simulink model "test_on_proxy"  (R2025b)
settings: Solver=FixedStepAuto  StartTime=0.0  StopTime=91  FixedStep=0.001  RelTol=1e-3
undefined symbols (not defined in the file): DiscIntNeverNeededParam, Ts, x0_eq
libraries: eeGeneralControl x1
(part 2 of 2)

== matlab function test_on_proxy/mpc_core_codegen2 ==
  data: theta_meas input; omega_meas input; eps_center_total_meas input; eps_center_dyn_meas input; theta_ref input; x_prev input; Jrig input; Brig input; max_angle input; Qth input; QtipVel input; Qbend input; Qq_base input; Qv_base input; umax input; du_rate_max input; Sdu input; Ru input; m_payload input; m_payload_step input; gravity_sign input; gravity_correction input; use_gravity_compensation input; zeta input; tol input; S_theta_base input; S_theta_high input; terminal_cost_gain_base input; terminal_law_gain_base input; term_gain_min input; term_gain_max input; S_term_box input; uNm output; u_mpc output; x_next output; y_geom output; y_rate output; EPS_my output; y_rate_mpc output; m_proj_base output; tau_g_ff output; offset_based_geom_angle output; terminal_cost_value output; terminal_error_norm output; terminal_u_lqr output; terminal_u_last output; terminal_u_match_error output; terminal_inside_flag output; terminal_lyap_delta output; terminal_cost_ratio output; alpha_term_vis output; terminal_cost_normalized output; terminal_inside_flag_strict output; terminal_inside_flag_soft output; terminal_set_slack output; terminal_set_box_violation output; z_out output; g_dyn output; x_hat output
function [uNm,u_mpc, x_next, y_geom, y_rate, EPS_my, y_rate_mpc, ...
          m_proj_base,tau_g_ff,offset_based_geom_angle, ...
          terminal_cost_value, terminal_error_norm, ...
          terminal_u_lqr, terminal_u_last, terminal_u_match_error, ...
          terminal_inside_flag, terminal_lyap_delta, ...
          terminal_cost_ratio, alpha_term_vis, ...
          terminal_cost_normalized, terminal_inside_flag_strict, terminal_inside_flag_soft, ...
          terminal_set_slack, terminal_set_box_violation,z_out,g_dyn,x_hat]  = mpc_core_codegen( ...
    theta_meas, omega_meas, ...
    eps_center_total_meas, ...
    eps_center_dyn_meas, ...
    theta_ref, x_prev,Jrig,Brig, ...
    max_angle,Qth,QtipVel,Qbend,Qq_base,Qv_base,umax,du_rate_max,Sdu,Ru,...
    m_payload,m_payload_step,gravity_sign,gravity_correction,use_gravity_compensation,...
    zeta,tol,S_theta_base,S_theta_high,...
    terminal_cost_gain_base,terminal_law_gain_base,term_gain_min,term_gain_max,S_term_box) %#codegen

NM = coder.const(1);                      % only 1 flex mode used
NX = coder.const(2 + 2*NM);              % x = [theta omega q v]
NY = coder.const(3 + 2*NM);              % y = [geom bend tiprate q v]
NP = coder.const(65);                    % prediction horizon
NC = coder.const(13);                    % control horizon
NS = coder.const(min(100, 60*NM));       % spatial integration points

Nm = NM; nx = NX; ny = NY; Np = NP; Nc = NC; Ns = NS;

persistent zeta_ref omega_ref init_zeta_ref
persistent last_m_payload_model

persistent L b  h E rho Izz EI Acs yb

persistent init_done
persistent Ts iy_geom iy_tipdot iy_bend
persistent m_beam
persistent g

persistent Ad Bd Taff Cd_static
persistent s Alpha aL dphiL Phi_hat rhoA Minv Minv_c
persistent Sx Su_base Su Qz w_trap

persistent u_prev dU_prev
persistent k_strain
persistent phi_tip_hat
persistent J_tip_eff

persistent buf_xa buf_yoff buf_Crow buf_q
persistent idx_qi idx_vi
persistent umax_stack dumax_vec

persistent pw_vec_ext
persistent max_iter

persistent theta_max
persistent M_con

persistent xnom_all Crow_all yoff_nom_all
persistent Fi_all Gi_all
persistent Gabs Ginc QGinc
persistent onesNc

persistent Pterm Kterm Cd_term0 Crow_term0
persistent alpha_term
persistent alpha_vis_scale
persistent theta_ref_clip_margin

persistent term_box

% --- persistents for total/dynamic epsilon handling ---
persistent q_total_filt_prev
persistent q_dyn_prev
persistent alpha_q_total
payload_step_eff = max(abs(m_payload_step), 1e-9);
if m_payload >= 0.1
   m_payload = 0; 
    
end
m_payload_model  = payload_step_eff * round(m_payload / payload_step_eff);

% ============================================================
% First-time fixed initialization
% ============================================================
if isempty(init_done)

  
    L   = 0.5;                            % beam length
    b   = 0.02;                           % beam width
    h   = 0.002;                          % beam thickness
    E   = 70e9;
    rho = 2755;
    Acs = b*h;
    Izz = b*h^3/12;
    EI  = E*Izz;
    rhoA = rho*Acs;                       % mass per length
    yb  = 0.5*h;                          % outer fiber distance for strain relation

    fs = 1000;
    Ts = 1/fs;

    g = 9.81;

     theta_max = max_angle * pi/180;
    M_con     = min(Np,15);
    max_iter  = 60;

    m_beam = rhoA * L;

    s = linspace(0,L,Ns).';

    w_trap = zeros(Ns,1);
    for i = 2:Ns
        hseg = s(i) - s(i-1);
        w_trap(i-1) = w_trap(i-1) + 0.5*hseg;
        w_trap(i)   = w_trap(i)   + 0.5*hseg;
    end

    iy_geom   = 1;
    iy_bend   = 2;
    iy_tipdot = 3;

    Qdiag = zeros(ny,1);
    Qdiag(iy_geom)   = Qth;
    Qdiag(iy_bend)   = Qbend;
    Qdiag(iy_tipdot) = QtipVel;

    rowQ = 3;
    for i = 1:Nm
        Qdiag(rowQ+i) = Qq_base;
    end

    rowV = 3 + Nm;
    for i = 1:Nm
        Qdiag(rowV+i) = Qv_base;
    end

    Qz = diag(Qdiag);

    u_prev  = 0;
    dU_prev = zeros(Nc,1);

    buf_xa   = zeros(nx,1);
    buf_yoff = zeros(ny,1);
    buf_Crow = zeros(1,nx);
    buf_q    = zeros(Nm,1);

    idx_qi = zeros(Nm,1);
    idx_vi = zeros(Nm,1);
    for i = 1:Nm
        idx_qi(i) = 2 + 2*(i-1) + 1;
        idx_vi(i) = idx_qi(i) + 1;
    end

    umax_stack = umax*ones(Nc,1);
    dumax_vec  = du_rate_max*ones(Nc,1);

    pw_vec_ext = ones(Nc+2,1) / sqrt(Nc+2);

    xnom_all      = zeros(nx,Np);
    Crow_all      = zeros(Np,nx);
    yoff_nom_all  = zeros(Np,1);
    Fi_all        = zeros(ny,Np);
    Gi_all        = zeros(ny,Nc,Np);

    Gabs  = zeros(ny,Nc);
    Ginc  = zeros(ny,Nc);
    QGinc = zeros(ny,Nc);

    onesNc = ones(Nc,1);

    alpha_vis_scale = 1.0;
    theta_ref_clip_margin = 0.5*pi/180.0;

    term_box = zeros(nx,1);
    term_box(1) = 40*pi/180.0;
    term_box(2) = 80*pi/180.0;
    term_box(3) = 1;
    term_box(4) = 1.0;

    q_dyn_prev         = 0.0;
    q_total_filt_prev  = 0.0;
    alpha_q_total      = 0.10;

    last_m_payload_model = -1e99;

    % =========================
    % NEW: initialize zeta reference
    % =========================
    init_zeta_ref = false;
    omega_ref = zeros(Nm,1);
    zeta_ref  = zeta;
end

% ============================================================
% Payload-dependent model rebuild
% ============================================================
if abs(m_payload_model - last_m_payload_model) > 1e-12 || isempty(init_done)

    M_phi   = m_payload_model;
    M_mass  = m_payload_model;
    M_betaL = m_payload_model;
    J_tip_eff = 0.0;

    betaL = compute_payload_roots(Nm, rhoA, EI, L, M_betaL, J_tip_eff);

    omega_n = zeros(Nm,1);
    scale_omega = sqrt(EI / rhoA) / (L^2);
    for i = 1:Nm
        omega_n(i) = (betaL(i)^2) * scale_omega;
    end

    z = zeros(Nm,1);

    Phi      = zeros(Ns,Nm);
    Alpha    = zeros(Ns,Nm);
    dphiL    = zeros(Nm,1);
    phi_tip_hat = zeros(Nm,1);

    for i = 1:Nm

        phi_raw  = payload_shape(betaL(i), L, s, rhoA, M_phi);
        dphi_raw = payload_shape_d(betaL(i), L, s, rhoA, M_phi);

        phi_tip = payload_shape(betaL(i), L, L, rhoA, M_phi);
        sc = 1 / max(abs(phi_tip), 1e-12);

        phi_raw  = phi_raw  * sc;
        dphi_raw = dphi_raw * sc;

        % =========================
        % Modal mass FULL
        % =========================
        m_eff_beam = dot(w_trap, rhoA*(phi_raw.^2));

        m_eff_payload = M_mass*(phi_raw(end)^2) ...
                      + J_tip_eff*(dphi_raw(end)^2);

        m_eff_total = m_eff_beam + m_eff_payload;

        % normalization
        cn = 1 / sqrt(max(m_eff_total,1e-12));

        % =========================
        % NEW: ZETA UPDATE WITH PAYLOAD
        % =========================
        % First model rebuild stores reference omega and zeta.
        % Later, when payload changes omega_n, zeta is updated so that:
        %
        %   2*zeta_new*omega_new = 2*zeta_ref*omega_ref
        %
        % This keeps the modal damping coefficient approximately constant.

        if ~init_zeta_ref
            zeta_ref  = zeta;
            omega_ref = omega_n;
            init_zeta_ref = true;
        end

        zeta_eff_i = zeta_ref * omega_ref(i) / max(omega_n(i),1e-12);

        % safety clamp
        zeta_eff_i = clamp_scalar(zeta_eff_i, 1e-5, 0.5);

        z(i) = zeta_eff_i;

        % =========================
        % STORE MODES
        % =========================
        Phi(:,i)       = phi_raw;
        Alpha(:,i)     = cn * dphi_raw;
        dphiL(i)       = cn * dphi_raw(end);
        phi_tip_hat(i) = cn * phi_raw(end);
    end

    Phi_hat = zeros(Ns,Nm);
    for i = 1:Nm
        phi_raw  = payload_shape(betaL(i), L, s, rhoA, M_phi);
        dphi_raw = payload_shape_d(betaL(i), L, s, rhoA, M_phi);
        phi_tip  = payload_shape(betaL(i), L, L, rhoA, M_phi);

        sc = 1 / max(abs(phi_tip), 1e-12);

        phi_raw  = phi_raw  * sc;
        dphi_raw = dphi_raw * sc;

        mi_loc = dot(w_trap, rhoA*(phi_raw.^2)) ...
               + M_mass*(phi_raw(end)^2) ...
               + J_tip_eff*(dphi_raw(end)^2);

        cn = 1 / sqrt(max(mi_loc,1e-12));

        Phi_hat(:,i)    = cn * phi_raw;
        Alpha(:,i)      = cn * dphi_raw;
        dphiL(i)        = cn * dphi_raw(end);
        phi_tip_hat(i)  = cn * phi_raw(end);
    end

    c_base = zeros(Nm,1);
    for i = 1:Nm
        c_base(i) = dot(w_trap, rhoA*(s .* Phi_hat(:,i))) ...
                  + M_mass * L * phi_tip_hat(i);
    end

    Mmod = eye(Nm);
    Kmod = diag(omega_n.^2);
    Dmod = diag(2*z(:).*omega_n(:));
    Minv = inv(Mmod);

    aL     = Alpha(end,:).';
    Minv_c = Minv * c_base;

    A = zeros(nx);
    B = zeros(nx,1);

    A(1,2) = 1;
    A(2,2) = -(Brig/Jrig);
    B(2,1) = 1/Jrig;

    Aqq = -Minv*Kmod;
    Avv = -Minv*Dmod;

    for i = 1:Nm
        qi = idx_qi(i);
        vi = idx_vi(i);

        A(qi,vi) = 1;

        for j = 1:Nm
            qj = idx_qi(j);
            vj = idx_vi(j);

            A(vi,qj) = A(vi,qj) + Aqq(i,j);
            A(vi,vj) = A(vi,vj) + Avv(i,j);
        end

        B(vi,1) = B(vi,1) - (1/Jrig)*Minv_c(i);
        A(vi,2) = A(vi,2) + (Brig/Jrig)*Minv_c(i);
    end

    [Ad,Bd,Taff] = c2d_expm_affine_vec(A,B,Ts);

    Cd_static = zeros(ny,nx);

    Cd_static(iy_tipdot,2) = 1;
    for i = 1:Nm
        vi = idx_vi(i);
        Cd_static(iy_tipdot,vi) = Cd_static(iy_tipdot,vi) + dphiL(i);
    end

    for i = 1:Nm
        qi = idx_qi(i);
        Cd_static(iy_bend,qi) = Cd_static(iy_bend,qi) + 1.0;
    end

    rowQ = 3;
    for i = 1:Nm
        Cd_static(rowQ+i, idx_qi(i)) = 1;
    end

    rowV = 3 + Nm;
    for i = 1:Nm
        Cd_static(rowV+i, idx_vi(i)) = 1;
    end

    [Sx,Su_base,Su] = precompute_prediction_scaffolds_fast(Ad,Bd,Np,Nc,nx);

    sensor_s = 0.05;
    k_strain = zeros(Nm,1);

    for i = 1:Nm
        phi_dd_i = payload_shape_dd(betaL(i), L, sensor_s, rhoA, M_phi);

        phi_tip  = payload_shape(betaL(i), L, L, rhoA, M_phi);
        sc       = 1 / max(abs(phi_tip), 1e-12);
        phi_dd_i = phi_dd_i * sc;

        dphi_raw = payload_shape_d(betaL(i), L, s, rhoA, M_phi) * sc;
        phi_raw  = payload_shape(betaL(i), L, s, rhoA, M_phi) * sc;

        mi_loc = dot(w_trap, rhoA*(phi_raw.^2)) ...
               + M_mass*(phi_raw(end)^2) ...
               + J_tip_eff*(dphi_raw(end)^2);

        cn = 1 / sqrt(max(mi_loc,1e-12));

        k_strain(i) = yb * cn * phi_dd_i;
    end

    xeq_term0 = zeros(nx,1);
    qtmp_term = zeros(Nm,1);
    Crow_tmp  = zeros(1,nx);

    [~, Crow_term0, ~] = chord_angle_and_jac_analytic( ...
        xeq_term0, Alpha, w_trap, Nm, qtmp_term, Crow_tmp);

    Cd_term0 = Cd_static;
    Cd_term0(iy_geom,:) = Crow_term0;

    Qx_term = zeros(nx,nx);
    Qx_term(1,1) = 1.0;
    Qx_term(2,2) = 0.5;
    Qx_term(3,3) = 0.2;
    Qx_term(4,4) = 0.1;

    [Pterm, Kterm] = dlqr_terminal_design_iter(Ad, Bd, Qx_term, max(Ru,1e-3));

    u_term_max     = umax;
    theta_term_max = theta_max;

    denom_u = Kterm * (Pterm \ Kterm.');
    if denom_u < 1e-12
        denom_u = 1e-12;
    end
    alpha_u = (u_term_max^2) / denom_u;

    hth = Crow_term0;
    denom_th = hth * (Pterm \ hth.');
    if denom_th < 1e-12
        denom_th = 1e-12;
    end
    alpha_th = (theta_term_max^2) / denom_th;

    alpha_term = min(alpha_u, alpha_th);
    init_done = true;
    last_m_payload_model = m_payload_model;
end

terminal_cost_value    = 0.0;
terminal_error_norm    = 0.0;
terminal_u_lqr         = 0.0;
terminal_u_last        = 0.0;
terminal_u_match_error = 0.0;
terminal_inside_flag   = 0.0;
terminal_lyap_delta    = 0.0;
terminal_cost_ratio    = 0.0;
alpha_term_vis         = alpha_vis_scale * alpha_term;
terminal_cost_normalized = 0.0;
terminal_inside_flag_strict = 0.0;
terminal_inside_flag_soft   = 0.0;
terminal_set_slack = 0.0;
terminal_set_box_violation = 0.0;

% -------------------------------------------------------------------------
% STATE RECONSTRUCTION
% -------------------------------------------------------------------------
x_hat = x_prev;
x_hat(1) = theta_meas;
x_hat(2) = omega_meas;

if isempty(q_dyn_prev)
   q_dyn_prev = x_hat(3);
end

% dynamic epsilon -> dynamic q/v used by controller
q_dyn_meas = eps_center_dyn_meas / k_strain(1);
v_dyn_raw  = (q_dyn_meas - q_dyn_prev) / Ts;
q_dyn_prev = q_dyn_meas;

% total epsilon -> full-bend monitor only
q_total_meas = eps_center_total_meas / k_strain(1);
q_total_now  = (1.0 - alpha_q_total)*q_total_filt_prev + alpha_q_total*q_total_meas;

% IMPORTANT:
% Controller state must use consistent q and v.
% Do not mix total q with dynamic v.
x_hat(3) = q_total_meas;
x_hat(4) = -v_dyn_raw;

q_total_filt_prev = q_total_now;

buf_xa(:) = x_hat;
xa = buf_xa;

% reconstructed total strain monitor
EPS_my = k_strain(1) * q_total_now;

% use total epsilon-based bend proxy only for offset-based monitor
offset_theoretical = -(0.5^3*EPS_my)/(3*(0.5-0.05)*0.5*0.002) ...
                   + (0.5405*0.5^2*cos(xa(1)))/(24*70e9*0.02*0.002^3/12)*(0.5-4*0.05);

x_Hafsa = cos(xa(1)) - offset_theoretical*sin(xa(1));
y_Hafsa = sin(xa(1)) - offset_theoretical*cos(xa(1));
offset_based_geom_angle = atan2(y_Hafsa,x_Hafsa);

[thg, Crow_now, y_off_now] = chord_angle_and_jac_analytic( ...
    xa, Alpha, w_trap, Nm, buf_q, buf_Crow);

Cd_now = Cd_static;
Cd_now(iy_geom,:) = Crow_now;

yoff_now = buf_yoff;
yoff_now(:) = 0;
yoff_now(iy_geom) = y_off_now;

y_now      = Cd_now*xa + yoff_now;
y_rate_mpc = y_now(iy_tipdot);

theta_ref_eff = clamp_scalar(theta_ref, -(theta_max - theta_ref_clip_margin), (theta_max - theta_ref_clip_margin));

dist_theta = theta_max - abs(thg);
if dist_theta < 10*pi/180
    S_theta = S_theta_high;
else
    S_theta = S_theta_base;
end

% -------------------------------------------------------------------------
% TERMINAL TARGET
% use pure zero-flex terminal target because dynamic epsilon is dynamic-only
% -------------------------------------------------------------------------
xeq_term = zeros(nx,1);
xeq_term(1) = theta_ref_eff;
xeq_term(2) = 0.0;
xeq_term(3) = 0.0;
xeq_term(4) = 0.0;

[tau_eq_ff, ~] = gravity_torque_ff_from_state( ...
    xeq_term, s, Alpha, gravity_sign, g, rhoA, m_payload, Nm, idx_qi);

u_eq_term = tau_eq_ff * use_gravity_compensation + gravity_correction;
u_eq_term = clamp_scalar(u_eq_term, -umax, umax);

x_nom = xa;
for i = 1:Np
    [g_dyn_nom, ~, ~] = gravity_vector_from_state( ...
        x_nom, Alpha, aL, w_trap, rhoA, Phi_hat, phi_tip_hat, Minv, ...
        gravity_sign, g, m_payload, Nm, nx, idx_qi, idx_vi);

    x_nom = Ad*x_nom + Bd*u_prev + Taff*g_dyn_nom;
    xnom_all(:,i) = x_nom;

    [~, Crow_i, yoff_i] = chord_angle_and_jac_analytic( ...
        x_nom, Alpha, w_trap, Nm, buf_q, buf_Crow);

    Crow_all(i,:)     = Crow_i;
    yoff_nom_all(i,1) = yoff_i;
end

rowsN = (Np-1)*nx + (1:nx);
GxN   = Su_base(rowsN,1:Nc) * Su;
xNnom = xnom_all(:,Np);
eNnom = xNnom - xeq_term;

term_metric_nom = eNnom.' * Pterm * eNnom;
term_ratio_nom  = term_metric_nom / max(alpha_term,1e-12);

term_sched = 1.0 / (1.0 + term_ratio_nom);
term_sched = clamp_scalar(term_sched, term_gain_min, term_gain_max);

terminal_cost_gain = terminal_cost_gain_base * term_sched;
terminal_law_gain  = terminal_law_gain_base  * term_sched;

H_base = zeros(Nc,Nc);
f_base = zeros(Nc,1);

for i = 1:Np
    rows_x = (i-1)*nx + (1:nx);
    mi_h = min(i, Nc);

    Cd_i = Cd_static;
    Cd_i(iy_geom,:) = Crow_all(i,:);

    Fi = Cd_i * xnom_all(:,i);

    Gabs(:,:) = Cd_i * Su_base(rows_x,1:Nc);
    Ginc(:,:) = Gabs * Su;

    for k = 1:Nc
        if k > mi_h
            for r = 1:ny
                Ginc(r,k) = 0;
            end
        end
    end

    QGinc(:,:) = Qz * Ginc;
    H_base = H_base + Ginc.' * QGinc;

    yi = Fi;
    yi(iy_geom) = yi(iy_geom) + yoff_nom_all(i) - theta_ref_eff;

    f_base = f_base + Ginc.' * (Qz * yi);

    Fi_all(:,i)   = Fi;
    Gi_all(:,:,i) = Ginc;
end

H_base = H_base + terminal_cost_gain * (GxN.' * Pterm * GxN);
f_base = f_base + terminal_cost_gain * (GxN.' * (Pterm * eNnom));

Su_last = zeros(1,Nc);
for k = 1:Nc
    Su_last(k) = 1.0;
end

a_term = Su_last - Kterm * GxN;
b_term = (Kterm * eNnom) + u_eq_term - u_prev;

H_base = H_base + terminal_law_gain * (a_term.' * a_term);
f_base = f_base - terminal_law_gain * (a_term.' * b_term);

H_base = H_base + (Ru * (Su.' * Su)) + Sdu*eye(Nc);
f_base = f_base + Ru * (Su.' * (u_prev * onesNc));

H_base = 0.5*(H_base + H_base.');

nU         = Nc;
nSlackAng  = 1;
nSlackTerm = 1;
nZ         = nU + nSlackAng + nSlackTerm;

idx_ang_slack  = nU + 1;
idx_term_slack = nU + 2;

H_ext = zeros(nZ,nZ);
H_ext(1:nU,1:nU) = H_base;
H_ext(idx_ang_slack,idx_ang_slack)  = 2*S_theta;
H_ext(idx_term_slack,idx_term_slack)= 2*S_term_box;

f_ext       = zeros(nZ,1);
f_ext(1:nU) = f_base;

Nlin   = 2*M_con + 1 + 2*nx + 1;
A_ineq = zeros(Nlin, nZ);
b_ineq = zeros(Nlin, 1);
row_idx = 0;

for i = 1:M_con
    Fi_i   = Fi_all(:,i);
    Gi_i   = Gi_all(:,:,i);
    yoff_i = yoff_nom_all(i);

    f_th_eff = Fi_i(iy_geom) + yoff_i;
    g_th     = Gi_i(iy_geom,:);

    row_up = zeros(1,nZ);
    row_up(1:nU) = g_th;
    row_up(idx_ang_slack) = -1;
    b_up = theta_max - f_th_eff;

    row_lo = zeros(1,nZ);
    row_lo(1:nU) = -g_th;
    row_lo(idx_ang_slack) = -1;
    b_lo = theta_max + f_th_eff;

    row_idx = row_idx + 1;
    A_ineq(row_idx,:) = row_up;
    b_ineq(row_idx)   = b_up;

    row_idx = row_idx + 1;
    A_ineq(row_idx,:) = row_lo;
    b_ineq(row_idx)   = b_lo;
end

row_idx = row_idx + 1;
A_ineq(row_idx,:)            = 0;
A_ineq(row_idx,idx_ang_slack)= -1;
b_ineq(row_idx)              = 0;

for j = 1:nx
    row_idx = row_idx + 1;
    A_ineq(row_idx,1:nU)          = GxN(j,:);
    A_ineq(row_idx,idx_term_slack)= -1;
    b_ineq(row_idx)               = term_box(j) - eNnom(j);

    row_idx = row_idx + 1;
    A_ineq(row_idx,1:nU)          = -GxN(j,:);
    A_ineq(row_idx,idx_term_slack)= -1;
    b_ineq(row_idx)               = term_box(j) + eNnom(j);
end

row_idx = row_idx + 1;
A_ineq(row_idx,:)             = 0;
A_ineq(row_idx,idx_term_slack)= -1;
b_ineq(row_idx)               = 0;

[Lips_ext, pw_vec_ext] = eigmax_local(H_ext, pw_vec_ext);
alpha_pg = 0.1/(Lips_ext + 1e-12);

if all(dU_prev==0)
    z0 = zeros(nZ,1);
else
    dU0 = zeros(Nc,1);
    dU0(1:end-1) = dU_prev(2:end);
    dU0(end)     = dU_prev(end);
    z0           = zeros(nZ,1);
    z0(1:nU)     = dU0;
end

z = projected_gradient_QP_lin_ineq_ext(H_ext,f_ext,z0, ...
                                       u_prev,Su,umax_stack,dumax_vec, ...
                                       A_ineq,b_ineq, ...
                                       alpha_pg,max_iter,tol,nU);
if ~all(isfinite(z))
    z = zeros(nZ,1);
end

dU = z(1:nU);
dU_prev = dU;

terminal_set_slack = z(idx_term_slack);
if ~isfinite(terminal_set_slack)
    terminal_set_slack = 0.0;
end

du    = dU(1);
u_mpc = clamp_scalar(u_prev + du, -umax, umax);

xN_pred = xNnom + GxN * dU;
eN_pred = xN_pred - xeq_term;

terminal_cost_value = eN_pred.' * Pterm * eN_pred;               % raw ellipsoidal cost
terminal_error_norm = sqrt(max(eN_pred.' * eN_pred, 0.0));       % plain Euclidean error norm

terminal_u_lqr  = u_eq_term + Kterm * eN_pred;
terminal_u_last = u_prev + sum(dU);
terminal_u_match_error = terminal_u_last - terminal_u_lqr;

alpha_term_vis = alpha_vis_scale * alpha_term;

% -----------------------------------------------------------------
% Robust terminal checking:
% 1) keep ellipsoidal metric only as secondary diagnostic
% 2) use normalized terminal box as main practical inside/outside test
% -----------------------------------------------------------------

% Ellipsoidal monitor only (can be badly scaled depending on Pterm/Qx_term)
terminal_cost_ratio = terminal_cost_value / max(alpha_term,1e-6);
terminal_cost_normalized = sqrt(max(terminal_cost_ratio,0.0));

% Box-normalized metric (much more interpretable)
box_norm_max = 0.0;
for j = 1:nx
    denom_j = max(term_box(j), 1e-9);
    rj = abs(eN_pred(j)) / denom_j;
    if rj > box_norm_max
        box_norm_max = rj;
    end
end

% strict / soft practical flags from box metric
if box_norm_max <= 1.0
    terminal_inside_flag_strict = 1.0;
else
    terminal_inside_flag_strict = 0.0;
end

if box_norm_max <= 1.5
    terminal_inside_flag_soft = 1.0;
else
    terminal_inside_flag_soft = 0.0;
end

terminal_inside_flag = terminal_inside_flag_soft;

% Terminal Lyapunov diagnostic must use the same affine gravity structure
% as the real model.
[g_dyn_tail, ~, ~] = gravity_vector_from_state( ...
    xN_pred, Alpha, aL, w_trap, rhoA, Phi_hat, phi_tip_hat, Minv, ...
    gravity_sign, g, m_payload, Nm, nx, idx_qi, idx_vi);

xNp1_tail = Ad * xN_pred + Bd * terminal_u_lqr + Taff*g_dyn_tail;
eNp1_tail = xNp1_tail - xeq_term;
terminal_lyap_delta = eNp1_tail.' * Pterm * eNp1_tail - terminal_cost_value;

terminal_set_box_violation = 0.0;
for j = 1:nx
    vj = abs(eN_pred(j)) - (term_box(j) + terminal_set_slack);
    if vj > terminal_set_box_violation
        terminal_set_box_violation = vj;
    end
end
terminal_set_box_violation = max(terminal_set_box_violation, 0.0);

[g_dyn, ~, psi_tip] = gravity_vector_from_state( ...
    xa, Alpha, aL, w_trap, rhoA, Phi_hat, phi_tip_hat, Minv, ...
    gravity_sign, g, m_payload, Nm, nx, idx_qi, idx_vi);

[tau_g_ff, psi_tip] = gravity_torque_ff_from_state( ...
    xa, s, Alpha, gravity_sign, g, rhoA, m_payload, Nm, idx_qi);

tau_g_ff = tau_g_ff * use_gravity_compensation;

u_unsat = u_mpc + tau_g_ff + gravity_correction;
uNm     = clamp_scalar(u_unsat, -umax, umax);
u_prev  = uNm;

x_next = Ad*xa + Bd*uNm + Taff * g_dyn;

% Recompute nonlinear output at x_next instead of using old linearization.
[~, Crow_next, yoff_next_geom] = chord_angle_and_jac_analytic( ...
    x_next, Alpha, w_trap, Nm, buf_q, buf_Crow);

Cd_next = Cd_static;
Cd_next(iy_geom,:) = Crow_next;

yoff_next = buf_yoff;
yoff_next(:) = 0;
yoff_next(iy_geom) = yoff_next_geom;

z_out  = Cd_next*x_next + yoff_next;
y_rate = z_out(iy_tipdot);

y_geom = thg;

m_proj_base = (m_payload + m_beam) * cos(psi_tip);
end


function val = eNpred_safe(Pterm, eN_pred)
val = Pterm * eN_pred;
end


function lambda_vec = compute_payload_roots(Nm, rhoA, EI, L, M_tip, J_tip)
lambda_vec = zeros(Nm,1);

cf_guess = [1.875104068711961; 4.694091132974174; 7.854757438237612; 10.995540734875466];

n_found = 0;
step = 0.05;
x_prev = 0.10;
f_prev = freq_eq_payload_lambda(x_prev, rhoA, L, M_tip, J_tip);

x = x_prev + step;
while (x <= 40.0) && (n_found < Nm)
    f_now = freq_eq_payload_lambda(x, rhoA, L, M_tip, J_tip);

    if isfinite(f_prev) && isfinite(f_now)
        if f_prev == 0
            n_found = n_found + 1;
            lambda_vec(n_found) = x_prev;
        elseif (f_prev * f_now) < 0
            n_found = n_found + 1;
            lambda_vec(n_found) = bisect_root_payload(x_prev, x, rhoA, L, M_tip, J_tip);
        end
    end

    x_prev = x;
    f_prev = f_now;
    x = x + step;
end

for k = n_found+1:Nm
    lambda_vec(k) = cf_guess(k);
end
end


function root = bisect_root_payload(a, b, rhoA, L, M_tip, J_tip)
fa = freq_eq_payload_lambda(a, rhoA, L, M_tip, J_tip);
fb = freq_eq_payload_lambda(b, rhoA, L, M_tip, J_tip);

if abs(fa) < 1e-12
    root = a;
    return;
end
if abs(fb) < 1e-12
    root = b;
    return;
end

for it = 1:80
    c = 0.5*(a+b);
    fc = freq_eq_payload_lambda(c, rhoA, L, M_tip, J_tip);

    if abs(fc) < 1e-12 || abs(b-a) < 1e-10
        root = c;
        return;
    end

    if (fa*fc) < 0
        b = c;
        fb = fc;
    else
        a = c;
        fa = fc;
    end
end

root = 0.5*(a+b);
end


function val = freq_eq_payload_lambda(lam, rhoA, L, M_tip, J_tip)
mu = 0.0;
den_m = rhoA * L;
if den_m > 1e-18
    mu = M_tip / den_m;
end

nu = 0.0;
den_j = rhoA * (L^3);
if den_j > 1e-18
    nu = J_tip / den_j;
end

c  = cos(lam);
s  = sin(lam);
ch = cosh(lam);
sh = sinh(lam);

term1 = 1.0 + c*ch;
term2 = mu * lam   * (s*ch - c*sh);
term3 = nu * lam^3 * (s*ch + c*sh);
term4 = mu * nu * lam^4 * (1.0 - c*ch);

val = term1 - term2 - term3 + term4;
end


function alpha = payload_alpha(lam, rhoA, L, M_tip)
a = 0.0;
den = rhoA * L;
if den > 1e-18
    a = M_tip / den;
end

num = sinh(lam) - sin(lam) + a*lam*(cosh(lam) - cos(lam));
dena = cos(lam) + cosh(lam) + a*lam*(sinh(lam) - sin(lam));

if abs(dena) < 1e-12
    dena = sign_nonzero(dena) * 1e-12;
end

alpha = num / dena;
end


function phi = payload_shape(betaL,L,s,rhoA,M_tip)
bs  = (betaL/L).*s;
alp = payload_alpha(betaL, rhoA, L, M_tip);
phi = cosh(bs) - cos(bs) + alp*(sin(bs) - sinh(bs));
end


function dphi = payload_shape_d(betaL,L,s,rhoA,M_tip)
bs  = (betaL/L).*s;
alp = payload_alpha(betaL, rhoA, L, M_tip);
dphi = (betaL/L) * (sinh(bs) + sin(bs) + alp*(cos(bs) - cosh(bs)));
end


function d2phi = payload_shape_dd(betaL,L,s,rhoA,M_tip)
bs  = (betaL/L).*s;
alp = payload_alpha(betaL, rhoA, L, M_tip);

% Correct second derivative of:
% phi = cosh(bs) - cos(bs) + alpha*(sin(bs) - sinh(bs))
d2phi = (betaL/L)^2 * (cosh(bs) + cos(bs) - alp*(sin(bs) + sinh(bs)));
end


function y = sign_nonzero(x)
if x >= 0
    y = 1.0;
else
    y = -1.0;
end
end


function [P,K] = dlqr_terminal_design_iter(A,B,Q,R)
n = size(A,1);
P = Q;

for it = 1:300
    S = R + B.'*P*B;
    if abs(S) < 1e-12
        S = sign_nonzero(S) * 1e-12;
    end

    K = -(S \ (B.'*P*A));
    Pn = Q + A.'*P*(A + B*K);

    Pn = 0.5*(Pn + Pn.');

    if norm(Pn - P, 'fro') < 1e-10 * (1 + norm(P, 'fro'))
        P = Pn;
        break;
    end
    P = Pn;
end

S = R + B.'*P*B;
if abs(S) < 1e-12
    S = sign_nonzero(S) * 1e-12;
end
K = -(S \ (B.'*P*A));

P = 0.5*(P + P.');
for i = 1:n
    P(i,i) = P(i,i) + 1e-10;
end
end


function [Ad,Bd,Taff] = c2d_expm_affine_vec(A,B,Ts)
n = size(A,1); m = size(B,2);
Blk = [A, B, eye(n); zeros(m,n+m+n); zeros(n,n+m+n)];
Ed  = expm(Blk*Ts);
Ad  = Ed(1:n,1:n);
Bd  = Ed(1:n,n+1:n+m);
Taff= Ed(1:n,n+m+1:n+m+n);
end


function [Sx,Su_base,Su] = precompute_prediction_scaffolds_fast(Ad,Bd,Np,Nc,nx)
Sx = zeros(Np*nx, nx);

A_pow = eye(nx);
for i = 1:Np
    A_pow = Ad*A_pow;
    Sx((i-1)*nx+(1:nx),:) = A_pow;
end

Su_base = zeros(Np*nx, Nc);
for j = 1:Nc
    row = j;
    blk = Bd;
    Su_base((row-1)*nx+(1:nx), j) = blk;
    for i = row+1:Np
        blk = Ad * blk;
        Su_base((i-1)*nx+(1:nx), j) = blk;
    end
end

Su = tril_ones(Nc);
end


function T = tril_ones(N)
T = zeros(N,N);
for i = 1:N
    for j = 1:i
        T(i,j)=1;
    end
end
end


function [theta_geom, Crow, y1_off] = chord_angle_and_jac_analytic( ...
    x_state, Alpha, w_trap, NM, q_buf, Crow_buf)

Crow = Crow_buf; Crow(:) = 0;

th = x_state(1);
for i = 1:NM
    q_buf(i) = x_state(2 + 2*(i-1) + 1);
end

psi  = th + Alpha*q_buf;
cpsi = cos(psi);
spsi = sin(psi);

xt = w_trap.' * cpsi;
yt = w_trap.' * spsi;

theta_geom = atan2(yt, xt);

D = xt*xt + yt*yt;
if D < 1e-12
    D = 1e-12;
end

Crow(1) = 1.0;
for i = 1:NM
    qi_idx = 2 + 2*(i-1) + 1;
    Ic = w_trap.' * (cpsi .* Alpha(:,i));
    Is = w_trap.' * (spsi .* Alpha(:,i));
    Crow(qi_idx) = (xt*Ic + yt*Is) / D;
end

y1_off = theta_geom - Crow * x_state(:);
end


function [g_dyn, a_grav_1, psi_tip] = gravity_vector_from_state( ...
    x_state, Alpha, aL, w_trap, rhoA, Phi_hat, phi_tip_hat, Minv, ...
    gravity_sign, g, m_payload, Nm, nx, idx_qi, idx_vi)

q = zeros(Nm,1);
for i = 1:Nm
    q(i) = x_state(idx_qi(i));
end

psi_tip = x_state(1) + (aL.' * q);

psi_s = x_state(1) + Alpha*q;
cpsi  = cos(psi_s);
cpsi_tip = cos(psi_tip);

w_now = zeros(1,Nm);
for j = 1:Nm
    w_now(1,j) = dot(w_trap, (rhoA * cpsi) .* Phi_hat(:,j)) ...
               + m_payload * cpsi_tip * phi_tip_hat(j);
end

a_beam = gravity_sign * g * (Minv * w_now.');

g_dyn = zeros(nx,1);
for i = 1:Nm
    g_dyn(idx_vi(i)) = g_dyn(idx_vi(i)) + a_beam(i);
end

a_grav_1 = a_beam(1);
end


function [tau_g_ff, psi_tip] = gravity_torque_ff_from_state( ...
    x_state, s, Alpha, gravity_sign, g, rhoA, m_payload, Nm, idx_qi)

q = zeros(Nm,1);
for i = 1:Nm
    q(i) = x_state(idx_qi(i));
end

psi  = x_state(1) + Alpha*q;
cpsi = cos(psi);

Ns = length(s);

x_pos = zeros(Ns,1);
for k = 2:Ns
    ds = s(k) - s(k-1);
    x_pos(k) = x_pos(k-1) + 0.5*ds*(cpsi(k-1) + cpsi(k));
end

x_tip   = x_pos(end);
psi_tip = psi(end);

tau_beam = 0;
for k = 2:Ns
    ds = s(k) - s(k-1);
    tau_beam = tau_beam + 0.5*ds * rhoA * (x_pos(k-1) + x_pos(k));
end
tau_beam = gravity_sign * g * tau_beam;

tau_payload = gravity_sign * g * m_payload * x_tip;

tau_g_ff = tau_beam + tau_payload;
end


function y = clamp_scalar(x,a,b)
y = min(max(x,a),b);
end


function [L, xw_out] = eigmax_local(H,xw_in)
x = xw_in;
ss = x.'*x;
if ss < 1e-18
    n = size(H,1);
    x = ones(n,1)/sqrt(n);
end
for k = 1:8
    x = H*x;
    nrm = sqrt(x'*x);
    if nrm < 1e-18
        break;
    end
    x = x/nrm;
end
xw_out = x;
L = (x'*(H*x))/(x'*x);
end


function z = projected_gradient_QP_lin_ineq_ext(H,f,z,u_prev,Su,umax_stack,dumax_vec, ...
                                                A_ineq,b_ineq,alpha,max_it,tol,Nc)

nZ = numel(z);

% ============================================================
% Build hard constraints for dU and absolute U
%
% dU <= dumax
% -dU <= dumax
%
% u_prev + Su*dU <= umax
% -(u_prev + Su*dU) <= umax
% ============================================================

nHard = 4*Nc;
A_hard = zeros(nHard,nZ);
b_hard = zeros(nHard,1);

row = 0;

% ---- delta-u upper/lower bounds
for k = 1:Nc
    row = row + 1;
    A_hard(row,k) = 1.0;
    b_hard(row)   = dumax_vec(k);

    row = row + 1;
    A_hard(row,k) = -1.0;
    b_hard(row)   = dumax_vec(k);
end

% ---- absolute-u upper/lower bounds
for k = 1:Nc
    row = row + 1;
    A_hard(row,1:Nc) = Su(k,:);
    b_hard(row)      = umax_stack(k) - u_prev;

    row = row + 1;
    A_hard(row,1:Nc) = -Su(k,:);
    b_hard(row)      = umax_stack(k) + u_prev;
end

% ============================================================
% Projected-gradient iterations
% ============================================================

for it = 1:max_it

    z_old = z;

    % ---- gradient step
    g = H*z + f;
    z_new = z - alpha*g;

    % ========================================================
    % Projection onto hard constraints
    % Sequential hyperplane projection:
    %
    % if a*z > b:
    % z = z - ((a*z-b)/(a*a'))*a'
    %
    % This is cleaner than simple clipping because all hard
    % inequalities are represented explicitly as A*z <= b.
    % ========================================================

    for sweep = 1:3
        for j = 1:nHard
            aj = A_hard(j,:);
            bj = b_hard(j);

            val = aj*z_new;

            if val > bj
                denom = aj*aj.';
                if denom > 1e-18
                    z_new = z_new - ((val - bj)/denom)*aj.';
                end
            end
        end
    end

    % ========================================================
    % Projection onto soft angle / terminal inequalities
    % These include slack variables, so they remain soft because
    % slack is penalized in H_ext.
    % ========================================================

    [m_con,~] = size(A_ineq);

    for sweep = 1:3
        for j = 1:m_con
            aj = A_ineq(j,:);
            bj = b_ineq(j);

            val = aj*z_new;

            if val > bj
                denom = aj*aj.';
                if denom > 1e-18
                    z_new = z_new - ((val - bj)/denom)*aj.';
                end
            end
        end
    end

    % ---- safety check
    if ~all(isfinite(z_new))
        z_new = z_old;
        break;
    end

    % ---- stopping condition
    step_norm = 0.0;
    for k = 1:nZ
        step_norm = step_norm + (z_new(k) - z(k))^2;
    end

    z = z_new;

    if step_norm < (0.1*tol)^2
        break;
    end

    if (g.'*g) < tol^2
        break;
    end
end

end


function x = backsolve_tril_ones(b)
n = numel(b);
x = zeros(n,1);
for i = 1:n
    s = 0.0;
    for j = 1:i-1
        s = s + x(j);
    end
    x(i) = b(i) - s;
end
end

== matlab function test_on_proxy/MATLAB Function7 ==
  data: t input; theta_ref output; theta_vec input; t0 input; Tr input; Twait input
    function theta_ref = multi_stage_ref(t, theta_vec, t0, Tr, Twait) %#codegen
    % MULTI-STAGE LINEAR RAMP REFERENCE (vector-based, codegen friendly)
    %
    % Sequence:
    %   Start from 0 rad
    %   Ramp to theta_vec(1) over Tr
    %   Wait Twait
    %   Ramp to theta_vec(2) over Tr
    %   Wait Twait
    %   ...
    %   Ramp to theta_vec(N) over Tr
    %   Hold theta_vec(N) forever
    %
    % Inputs:
    %   t         : current time [s]
    %   theta_vec : [Nx1] or [1xN] vector of target angles [rad]
    %   t0        : start time of first ramp [s]
    %   Tr        : ramp duration for ALL ramps [s]
    %   Twait     : wait duration BETWEEN ramps [s]
    %
    % Output:
    %   theta_ref : scalar reference at time t
    
    n = length(theta_vec);
    
    % If empty vector, stay at zero
    if n <= 0
        theta_ref = 0.0;
        return;
    end
    
    % Before first ramp: stay at zero
    if t < t0
        theta_ref = 0.0;
        return;
    end
    
    % Walk through all target segments
    prev_theta = 0.0;
    seg_start  = t0;
    
    for k = 1:n
        curr_theta = theta_vec(k);
    
        ramp_start = seg_start;
        ramp_end   = ramp_start + Tr;
    
        % ----- Ramp prev_theta -> curr_theta -----
        if t <= ramp_end
            s = (t - ramp_start) / Tr;
            if s < 0
                s = 0;
            elseif s > 1
                s = 1;
            end
            theta_ref = prev_theta + (curr_theta - prev_theta) * s;
            return;
        end
    
        % ----- After last ramp: hold forever -----
        if k == n
            theta_ref = curr_theta;
            return;
        end
    
        wait_end = ramp_end + Twait;
    
        % ----- Hold curr_theta before next ramp -----
        if t <= wait_end
            theta_ref = curr_theta;
            return;
        end
    
        % Move to next segment
        prev_theta = curr_theta;
        seg_start  = wait_end;
    end
    
    % Fallback: hold last target
    theta_ref = theta_vec(n);
    end
